simulink model "makshud_lab"  (R2024b)
settings: Solver=VariableStepAuto  StartTime=0.0  StopTime=0.05  RelTol=1e-3
undefined symbols (not defined in the file or in its folder): physconst
libraries: phasedenvlib x6, phasedtxrxlib x2, phasedwavlib x1, phaseddetectlib x1
settings Model: Creator=jahid  LastModifiedBy=mrmak
settings DataIOCC: ReturnWorkspaceOutputs=off

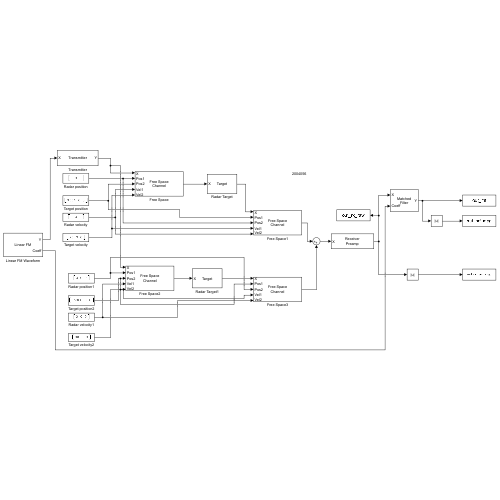
[thumbnail: Simulink's stored preview of the top-level diagram]
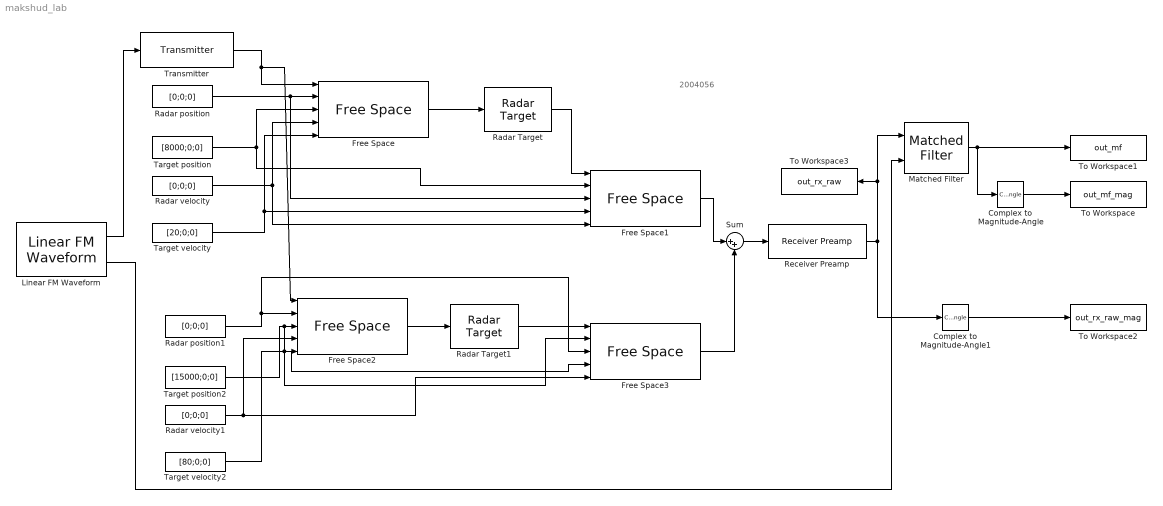
== system makshud_lab ==
  note: 2004056
  Complex to Magnitude-Angle : ComplexToMagnitudeAngle  Output=Magnitude
  Complex to Magnitude-Angle1 : ComplexToMagnitudeAngle  Output=Magnitude
  Free Space{,1..3} (4 alike) : phasedenvlib/Free Space  PropagationSpeed=physconst( 'LightSpeed' )  OperatingFrequency=5e9  TwoWayPropagation=off  SampleRateFromInputCheckbox=on  SampleRate=1e6  MaximumDistanceSource=Property  MaximumDistance=20e3  MaximumNumInputSamplesSource=Auto  MaximumNumInputSamples=1000  SimulateUsing=Interpreted execution
  Linear FM Waveform : phasedwavlib/Linear FM Waveform  SampleRate=12e6  DurationSpecification=Pulse width  PulseWidth=20e-6  DutyCycle=0.5  PRF=6000  PRFSelectionInputPort=off  SimulationTimeSource=Derive from waveform parameters  SweepBandwidth=3e6  SweepDirection=Up  SweepInterval=Positive  Envelope=Rectangular  FrequencyOffsetSource=Property  FrequencyOffset=0  OutputFormat=Pulses  NumSamples=100  NumPulses=1  PRFOutputPort=off  CoefficientsOutputPort=on  SimulateUsing=Interpreted execution
  Matched Filter : phaseddetectlib/Matched Filter  CoefficientsSource=Input port  Coefficients=[ 1; 1 ]  SpectrumWindow=None  CustomSpectrumWindow=@hamming  SpectrumRange=[ 0, 1e5 ]  SampleRateFromInputCheckbox=on  SampleRate=1e6  SidelobeAttenuation=30  Beta=0.5  Nbar=4  GainOutputPort=off  MaximumNumInputSamplesSource=Auto  MaximumNumInputSamples=100  SimulateUsing=Interpreted execution
  Radar Target : phasedenvlib/Radar Target  EnablePolarization=off  Mode=Monostatic  MeanRCSSource=Property  ScatteringMatrixSource=Property  MeanRCS=1000  ScatteringMatrix=eye( 2 )  Model=Nonfluctuating  PropagationSpeed=physconst( 'LightSpeed' )  OperatingFrequency=5e9  SeedSource=Auto  Seed=0  SimulateUsing=Interpreted execution
  Radar Target1 : phasedenvlib/Radar Target  EnablePolarization=off  Mode=Monostatic  MeanRCSSource=Property  ScatteringMatrixSource=Property  MeanRCS=100000  ScatteringMatrix=eye( 2 )  Model=Nonfluctuating  PropagationSpeed=physconst( 'LightSpeed' )  OperatingFrequency=5e9  SeedSource=Auto  Seed=0  SimulateUsing=Interpreted execution
  Radar position : Constant  Value=[0;0;0]
  Radar position1 : Constant  Value=[0;0;0]
  Radar velocity : Constant  Value=[0;0;0]
  Radar velocity1 : Constant  Value=[0;0;0]
  Receiver Preamp : phasedtxrxlib/Receiver Preamp  Gain=20  LossFactor=0  NoiseMethod=Noise temperature  NoiseFigure=0  ReferenceTemperature=290  SampleRateFromInputCheckbox=on  SampleRate=1e6  NoisePower=0  EnableInputPort=off  PhaseNoiseInputPort=off  SeedSource=Auto  Seed=0  SimulateUsing=Interpreted execution
  Sum : Sum  Inputs=|++
  Target position : Constant  Value=[8000;0;0]
  Target position2 : Constant  Value=[15000;0;0]
  Target velocity : Constant  Value=[20;0;0]
  Target velocity2 : Constant  Value=[80;0;0]
  To Workspace : ToWorkspace  VariableName=out_mf_mag  SampleTime=-1
  To Workspace1 : ToWorkspace  VariableName=out_mf  SampleTime=-1
  To Workspace2 : ToWorkspace  VariableName=out_rx_raw_mag  SampleTime=-1
  To Workspace3 : ToWorkspace  VariableName=out_rx_raw  SampleTime=-1
  Transmitter : phasedtxrxlib/Transmitter  PeakPower=50000  GainMethod=Linear  Gain=40  LossFactor=0  OIP3=Inf  Table=[ -25, 5, -1; -10, 20, -2; 0, 27, 12; 5, 28, 12 ]  InUseOutputPort=off  CoherentOnTransmit=on  PhaseNoiseOutputPort=off  SimulateUsing=Interpreted execution  NoiseMethod=None  NoiseFigure=3  NoiseFactor=2  NoiseTemperature=290  ReferenceTemperature=290  SampleRate=1e6  SampleRateFromInputCheckbox=on  PhaseOffset=0  SeedSource=Auto  Seed=0
  wires:
  Linear FM Waveform/1 -> Transmitter/1
  Transmitter/1 -> Free Space2/1, Free Space/1
  Radar position/1 -> Free Space1/3, Free Space/2
  Target position/1 -> Free Space/3, Free Space1/2
  Radar velocity/1 -> Free Space1/5, Free Space/4
  Target velocity/1 -> Free Space/5, Free Space1/4
  Free Space/1 -> Radar Target/1
  Complex to Magnitude-Angle/1 -> To Workspace/1
  Receiver Preamp/1 -> Matched Filter/1, To Workspace3/1, Complex to Magnitude-Angle1/1
  Matched Filter/1 -> To Workspace1/1, Complex to Magnitude-Angle/1
  Linear FM Waveform/2 -> Matched Filter/2
  Radar Target1/1 -> Free Space3/1
  Free Space2/1 -> Radar Target1/1
  Radar position1/1 -> Free Space3/3, Free Space2/2
  Target position2/1 -> Free Space3/2, Free Space2/3
  Radar velocity1/1 -> Free Space3/5, Free Space2/4
  Target velocity2/1 -> Free Space3/4, Free Space2/5
  Radar Target/1 -> Free Space1/1
  Free Space3/1 -> Sum/2
  Free Space1/1 -> Sum/1
  Sum/1 -> Receiver Preamp/1
  Complex to Magnitude-Angle1/1 -> To Workspace2/1
